simulink model "rctrigger"  (R2024a)
settings: Solver=VariableStepAuto  StartTime=0.0  StopTime=0.06  RelTol=1e-3
libraries: spsSeriesRLCBranchLib x5, spsVoltageMeasurementLib x4, spsACVoltageSourceLib x1, spsDiodeLib x1, spsThyristorLib x1, sps_lib x1
settings Model: Creator=Adithyan  LastModifiedBy=Adithyan
settings SolverCC: ZeroCrossAlgorithm=Adaptive
settings DebuggingCC: IgnoredZcDiagnostic=none

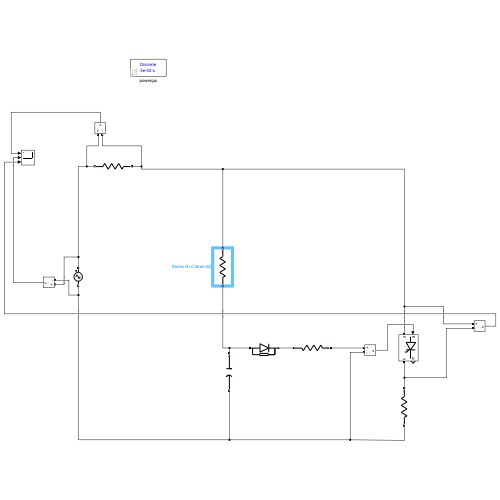
[thumbnail: Simulink's stored preview of the top-level diagram]
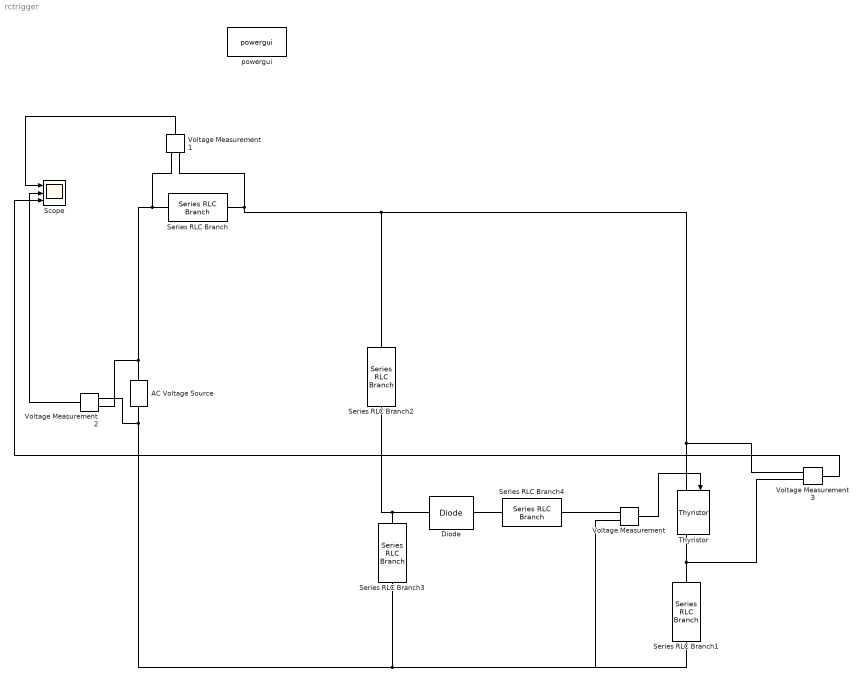
== system rctrigger ==
  AC Voltage Source : spsACVoltageSourceLib/AC Voltage Source  Amplitude=230*sqrt(2)  Phase=0  Frequency=60  SampleTime=0  Measurements=None  BusType=swing  Pref=10e3  Qref=0  Qmin=-inf  Qmax=+inf
  Diode : spsDiodeLib/Diode  Ron=0.001  Lon=0  Vf=0.8  IC=0  UseSnubber=0  Rs=500  Cs=0.1e-12  Measurements=off
  Scope : Scope  NumInputPorts=3
  Series RLC Branch : spsSeriesRLCBranchLib/Series RLC Branch  LConnTagsString=__new0  RConnTagsString=__new0  BranchType=R  Resistance=100  Inductance=1e-3  SetiL0=off  InitialCurrent=0  Capacitance=1e-6  Setx0=off  InitialVoltage=0  Measurements=None
  Series RLC Branch1 : spsSeriesRLCBranchLib/Series RLC Branch  LConnTagsString=__new0  RConnTagsString=__new0  BranchType=R  Resistance=10  Inductance=1e-3  SetiL0=off  InitialCurrent=0  Capacitance=1e-6  Setx0=off  InitialVoltage=0  Measurements=None
  Series RLC Branch2 : spsSeriesRLCBranchLib/Series RLC Branch  LConnTagsString=__new0  RConnTagsString=__new0  BranchType=R  Resistance=60e3  Inductance=1e-3  SetiL0=off  InitialCurrent=0  Capacitance=1e-6  Setx0=off  InitialVoltage=0  Measurements=None
  Series RLC Branch3 : spsSeriesRLCBranchLib/Series RLC Branch  LConnTagsString=__new0  RConnTagsString=__new0  BranchType=C  Resistance=500  Inductance=1e-3  SetiL0=off  InitialCurrent=0  Capacitance=1e-6  Setx0=off  InitialVoltage=0  Measurements=None
  Series RLC Branch4 : spsSeriesRLCBranchLib/Series RLC Branch  LConnTagsString=__new0  RConnTagsString=__new0  BranchType=R  Resistance=100  Inductance=1e-3  SetiL0=off  InitialCurrent=0  Capacitance=1e-6  Setx0=off  InitialVoltage=0  Measurements=None
  Thyristor : spsThyristorLib/Thyristor  Ron=0.001  Lon=0  Vf=0.8  IC=0  Rs=500  Cs=0  Measurements=on
  Voltage Measurement{,1..3} (4 alike) : spsVoltageMeasurementLib/Voltage Measurement  PhasorSimulation=off  OutputType=Complex  PSBequivalent=0
  powergui : sps_lib/powergui  Priority=1  SimulationMode=Discrete  SampleTime=50e-6  frequency=60  Iterations=50  frequencyindice=60  Pbase=100e6  ErrMax=1e-4  UnitsV=kV  UnitsW=MW  buscounter=0  FunctionMessages=off  echomessages=off  EnableUseOfTLC=off  CurrentSourceSwitches=off  DisableSnubberDevices=off  DisableRonSwitches=off  DisableVfSwitches=off  DisplayEquations=off  AutomaticDiscreteSolvers=off  SolverType=Tustin/Backward Euler (TBE)  Interpol=off  ExternalGateDelay=off  methode=off  Ts=100  x0status=blocks  SPID=on  SwTol=0  HookPort=off  NonlinearTolerance=1e-4  nMaxIteration=100  ContinueOnMaxIteration=off  RestoreLinks=warning  ResistiveCurrentMeasurement=off  Frange=[0:2:500]  Ylog=off  Xlog=on  ShowGrid=off  save=off  variable=ZData  structure=0  ZoomFFT=off  StartTime=0.0  cycles=1  DisplayStyle=1  fundamental=60  FreqAxis=off  MaxFrequency=1000  frequencyindicesteady=1  RmsSteady=1  display=off
  wires:
  Voltage Measurement2/1 -> Scope/2
  Voltage Measurement1/1 -> Scope/1
  Voltage Measurement/1 -> Thyristor/1
  Voltage Measurement3/1 -> Scope/3
  connections:
  Series RLC Branch/LConn1 -- Voltage Measurement1/LConn1 -- Voltage Measurement2/LConn1 -- AC Voltage Source/RConn1
  Series RLC Branch3/RConn1 -- Voltage Measurement2/LConn2 -- AC Voltage Source/LConn1 -- Series RLC Branch1/RConn1 -- Voltage Measurement/LConn2
  Diode/LConn1 -- Series RLC Branch2/RConn1 -- Series RLC Branch3/LConn1
  Thyristor/LConn1 -- Voltage Measurement3/LConn1 -- Series RLC Branch2/LConn1 -- Series RLC Branch/RConn1 -- Voltage Measurement1/LConn2
  Series RLC Branch4/LConn1 -- Voltage Measurement/LConn1
  Thyristor/RConn1 -- Voltage Measurement3/LConn2 -- Series RLC Branch1/LConn1
  Diode/RConn1 -- Series RLC Branch4/RConn1
